simulink model "Practical3_Cascaded_PD"  (R2026b)
settings: Solver=ode4  StopTime=15  FixedStep=0.01  MaxStep=0.01  RelTol=1e-6  AbsTol=1e-8
values from neighbouring files (symbols this model uses):
  A = [ones(1,4); -rotor_xy(2,:); rotor_xy(1,:); (kM/kT)*sigma(:).']    [practical3_setup.m]    (also in run_practical3_tests.m = reshape(ts.Data, [], numel(ts.Time)).')
  c_drag = 0    [practical2_parameters.m]    (also in practical3_setup.m)
  e0 = zeros(3,1)    [practical3_setup.m]
  e1 = e0    [practical3_setup.m]
  g = 9.81    [practical2_parameters.m]
  J = diag(Jdiag)    [practical2_parameters.m]
  Jdiag = [0.03;0.03;0.05]*(m0/1.5)*(l/0.25)^2    [practical2_parameters.m]
  kM = kMT*kT    [practical2_parameters.m]
  kT = 2*m_nom*g/(4*Omega_max^2)    [practical2_parameters.m]
  m = m_nom    [practical2_parameters.m]    (also in practical3_setup.m)
  m_nom = 1.50*m0    [practical2_parameters.m]
  mode = 2    [practical3_setup.m]    (also in run_practical3_tests.m)
  Omega_max = 800    [practical2_parameters.m]    (also in run_practical3_tests.m = 575)
  p0 = zeros(3,1)    [practical3_setup.m]
  p1 = p0    [practical3_setup.m]    (also in run_practical3_tests.m = [.50;.30;-.50];  e1(3) = 15*pi/180)
  rotor_xy = [d d -d -d; -d d d -d]    [practical2_parameters.m]
  sigma = [1;-1;1;-1]    [practical2_parameters.m]
  tiltMax = 20*pi/180    (= 0.349065850399)    [practical3_setup.m]
  wnAtt = 6    [practical3_setup.m]
  wnD = 1.00    (= 1)    [practical3_setup.m]
  wnXY = 0.70    (= 0.7)    [practical3_setup.m]
  X0 = zeros(12,1)    [practical2_parameters.m]
  zeta = 1.00    (= 1)    [practical3_setup.m]
settings Model: Creator=nicholas  LastModifiedBy=Nicholas Khor

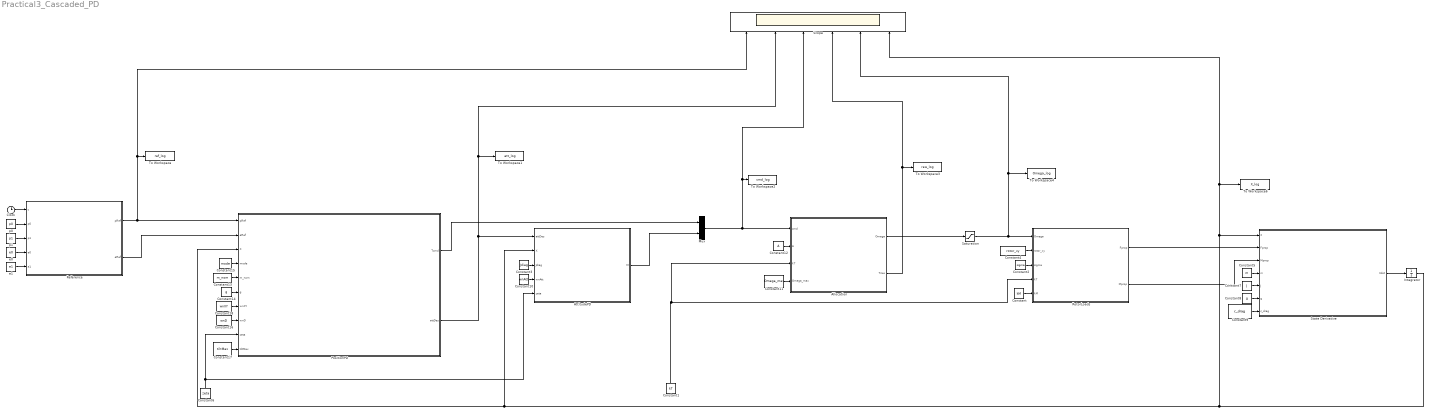
== system Practical3_Cascaded_PD ==
  Allocation : MATLAB Function  TreatAsAtomicUnit=on
  AttitudePD : MATLAB Function  TreatAsAtomicUnit=on
  Clock : Clock
  Constant : Constant  Value=kM
  Constant1 : Constant  Value=kT
  Constant10 : Constant  Value=wnAtt
  Constant11 : Constant  Value=Omega_max
  Constant12 : Constant  Value=A
  Constant13 : Constant  Value=m_nom
  Constant14 : Constant  Value=g
  Constant15 : Constant  Value=mode
  Constant16 : Constant  Value=wnD
  Constant17 : Constant  Value=tiltMax
  Constant18 : Constant  Value=wnXY
  Constant2 : Constant  Value=sigma
  Constant3 : Constant  Value=Jdiag
  Constant4 : Constant  Value=rotor_xy
  Constant5 : Constant  Value=m
  Constant6 : Constant  Value=zeta
  Constant7 : Constant  Value=J
  Constant8 : Constant  Value=g
  Constant9 : Constant  Value=c_drag
  Integrator : Integrator  InitialCondition=X0
  Mux : Mux  Inputs=2
  PositionPD : MATLAB Function  TreatAsAtomicUnit=on
  Reference : MATLAB Function  TreatAsAtomicUnit=on
  RotorLoads : MATLAB Function  TreatAsAtomicUnit=on
  Saturation : Saturate  UpperLimit=Omega_max  LowerLimit=0
  Scope : Scope  NumInputPorts=6
      settings: ActiveDisplayYMinimum=-105.17548172769591  ActiveDisplayYMaximum=797.29186581941735
  State Derivative : MATLAB Function  TreatAsAtomicUnit=on
  To Workspace : ToWorkspace  VariableName=ref_log  SaveFormat=Timeseries  SampleTime=-1
  To Workspace1 : ToWorkspace  VariableName=att_log  SaveFormat=Timeseries  SampleTime=-1
  To Workspace2 : ToWorkspace  VariableName=cmd_log  SaveFormat=Timeseries  SampleTime=-1
  To Workspace3 : ToWorkspace  VariableName=raw_log  SaveFormat=Timeseries  SampleTime=-1
  To Workspace4 : ToWorkspace  VariableName=Omega_log  SaveFormat=Timeseries  SampleTime=-1
  To Workspace6 : ToWorkspace  VariableName=X_log  SaveFormat=Timeseries  SampleTime=-1
  e0 : Constant  Value=e0
  e1 : Constant  Value=e1
  p0 : Constant  Value=p0
  p1 : Constant  Value=p1
  wires:
  Constant4/1 -> RotorLoads/2(rotor_xy)
  Constant2/1 -> RotorLoads/3(sigma)
  Constant/1 -> RotorLoads/5(kM)
  RotorLoads/1(Fprop) -> State Derivative/2(Fprop)
  RotorLoads/2(Mprop) -> State Derivative/3(Mprop)
  Constant5/1 -> State Derivative/4(m)
  Constant7/1 -> State Derivative/5(J)
  Constant8/1 -> State Derivative/6(g)
  Constant9/1 -> State Derivative/7(c_drag)
  State Derivative/1(Xdot) -> Integrator/1
  Integrator/1 -> PositionPD/3(X), AttitudePD/2(X), State Derivative/1(X), To Workspace6/1, Scope/6
  Clock/1 -> Reference/1(t)
  p0/1 -> Reference/2(p0)
  p1/1 -> Reference/3(p1)
  e0/1 -> Reference/4(e0)
  e1/1 -> Reference/5(e1)
  Constant6/1 -> AttitudePD/5(zeta), PositionPD/9(zeta)
  Constant10/1 -> AttitudePD/4(wnAtt)
  Constant3/1 -> AttitudePD/3(Jdiag)
  AttitudePD/1(M) -> Mux/2
  Mux/1 -> To Workspace2/1, Scope/3, Allocation/1(cmd)
  Constant11/1 -> Allocation/4(Omega_max)
  Constant12/1 -> Allocation/2(A)
  Allocation/1(Omega) -> Saturation/1
  Allocation/2(Traw) -> To Workspace3/1, Scope/4
  Reference/1(pRef) -> PositionPD/1(pRef), Scope/1, To Workspace/1
  Reference/2(eRef) -> PositionPD/2(eRef)
  PositionPD/1(Tcmd) -> Mux/1
  PositionPD/2(attDes) -> Scope/2, To Workspace1/1, AttitudePD/1(attDes)
  Constant14/1 -> PositionPD/6(g)
  Constant13/1 -> PositionPD/5(m_nom)
  Constant15/1 -> PositionPD/4(mode)
  Constant16/1 -> PositionPD/8(wnD)
  Constant18/1 -> PositionPD/7(wnXY)
  Constant17/1 -> PositionPD/10(tiltMax)
  Constant1/1 -> RotorLoads/4(kT), Allocation/3(kT)
  Saturation/1 -> RotorLoads/1(Omega), To Workspace4/1, Scope/5

== matlab function Practical3_Cascaded_PD/State Derivative ==
  data: X input; Xdot output; Fprop input; Mprop input; m input; J input; g input; c_drag input
function Xdot = StateDerivative(X,Fprop,Mprop,m,J,g,c_drag)
% Compute 12-state rigid-body quadrotor derivatives in NED / body axes.

% Extract states
vb    = X(4:6);
phi   = X(7);
theta = X(8);
psi   = X(9);
omega = X(10:12);

% Body-to-NED rotation matrix R = Rz * Ry * Rx
Rx = [1 0 0; 0 cos(phi) -sin(phi); 0 sin(phi) cos(phi)];
Ry = [cos(theta) 0 sin(theta); 0 1 0; -sin(theta) 0 cos(theta)];
Rz = [cos(psi) -sin(psi) 0; sin(psi) cos(psi) 0; 0 0 1];
R  = Rz * Ry * Rx;

% Position kinematics (NED)
pos_dot = R * vb;

% Translational dynamics (body axes)
Fg     = R.' * [0; 0; m*g];
Fdrag  = -c_drag * vb;
vb_dot = (Fg + Fprop + Fdrag)/m - cross(omega, vb);

% Attitude kinematics (Euler angle rates)
E = [1  sin(phi)*tan(theta)   cos(phi)*tan(theta);
    0  cos(phi)             -sin(phi);
    0  sin(phi)/cos(theta)   cos(phi)/cos(theta)];
euler_dot = E * omega;

% Rotational dynamics (body axes)
omega_dot = J \ (Mprop - cross(omega, J * omega));

% Assemble 12x1 state derivative
Xdot = zeros(12,1);
Xdot(1:3)   = pos_dot;
Xdot(4:6)   = vb_dot;
Xdot(7:9)   = euler_dot;
Xdot(10:12) = omega_dot;
end

== matlab function Practical3_Cascaded_PD/RotorLoads ==
  data: Omega input; Fprop output; rotor_xy input; sigma input; kT input; kM input; Mprop output
function [Fprop,Mprop] = RotorLoads(Omega,rotor_xy,sigma,kT,kM)
% Sum the thrust forces and moments from all 4 rotors in body axes
% (x forward, y right, z down).

Fprop = zeros(3,1);
Mprop = zeros(3,1);

for i = 1:4
    Ti = kT * Omega(i)^2;
    Fi = [0; 0; -Ti];
    ri = [rotor_xy(1,i); rotor_xy(2,i); 0];
    Mi = cross(ri, Fi) + [0; 0; sigma(i) * kM * Omega(i)^2];

    Fprop = Fprop + Fi;
    Mprop = Mprop + Mi;
end
end

== matlab function Practical3_Cascaded_PD/Reference ==
  data: t input; pRef output; p0 input; p1 input; e0 input; e1 input; eRef output
function [pRef, eRef] = Reference(t, p0, p1, e0, e1)
% Position: step from p0 to p1 at t = 1 s
if t < 1
    pRef = p0;
else
    pRef = p1;
end

% Attitude: smooth 1-second ramp (smoothstep) from e0 to e1, starting at t = 1 s
u = min(1, max(0, t - 1));
S = u^2 * (3 - 2*u);
eRef = e0 + S*(e1 - e0);

% Wrap the yaw reference to (-pi, pi]
eRef(3) = atan2(sin(eRef(3)), cos(eRef(3)));
end

== matlab function Practical3_Cascaded_PD/AttitudePD ==
  data: attDes input; M output; X input; Jdiag input; wnAtt input; zeta input
function M = AttitudePD(attDes, X, Jdiag, wnAtt, zeta)
att   = X(7:9);      % [phi; theta; psi]
rates = X(10:12);    % [p; q; r]

e = attDes - att;
e(3) = atan2(sin(e(3)), cos(e(3)));   % shortest-path yaw error

M = Jdiag(:) .* (wnAtt^2 * e - 2*zeta*wnAtt * rates);
end

== matlab function Practical3_Cascaded_PD/Allocation ==
  data: cmd input; Omega output; A input; kT input; Omega_max input; Traw output
function [Omega, Traw] = Allocation(cmd, A, kT, Omega_max)
% cmd = [Tcmd; Mx; My; Mz]
Traw     = A \ cmd;                       % requested rotor thrusts (may be infeasible)
Tmax     = kT*Omega_max^2;
Tbounded = min(Tmax, max(0, Traw));       % clip to [0, Tmax]
Omega    = sqrt(Tbounded/kT);
end

== matlab function Practical3_Cascaded_PD/PositionPD ==
  data: pRef input; Tcmd output; eRef input; X input; mode input; m_nom input; g input; wnXY input; wnD input; zeta input; tiltMax input; attDes output
function [Tcmd, attDes] = PositionPD(pRef, eRef, X, mode, m_nom, g, wnXY, wnD, zeta, tiltMax)
if mode == 1
    % Attitude-only: hover thrust, attitude straight from Reference
    Tcmd   = m_nom*g;
    attDes = eRef;
    return
end

phi = X(7); theta = X(8); psi = X(9);
p   = X(1:3);                         % [pN; pE; pD]

% Body velocity -> NED velocity (same R as Lab 2 StateDerivative)
Rx = [1 0 0; 0 cos(phi) -sin(phi); 0 sin(phi) cos(phi)];
Ry = [cos(theta) 0 sin(theta); 0 1 0; -sin(theta) 0 cos(theta)];
Rz = [cos(psi) -sin(psi) 0; sin(psi) cos(psi) 0; 0 0 1];
vNED = (Rz*Ry*Rx) * X(4:6);

% --- Vertical (Down) ---
aD = wnD^2*(pRef(3) - p(3)) - 2*zeta*wnD*vNED(3);
aD = min(0.5*g, max(-0.5*g, aD));
den  = max(cos(phi)*cos(theta), 0.5);           % guard against large tilt
Tcmd = m_nom*(g - aD)/den;

% --- Horizontal (North, East) ---
aN = wnXY^2*(pRef(1) - p(1)) - 2*zeta*wnXY*vNED(1);
aE = wnXY^2*(pRef(2) - p(2)) - 2*zeta*wnXY*vNED(2);

% Rotate NED acceleration into heading frame (yaw only)
aForward =  cos(psi)*aN + sin(psi)*aE;
aRight   = -sin(psi)*aN + cos(psi)*aE;

phiRef   = min(tiltMax, max(-tiltMax,  aRight/g));
thetaRef = min(tiltMax, max(-tiltMax, -aForward/g));

attDes = [phiRef; thetaRef; eRef(3)];
end
